simulink model "chip_route_circuit"  (R2025b)
settings: Solver=VariableStepAuto  StartTime=0.0  StopTime=10.0  RelTol=1e-3
libraries: fl_lib x44, nesl_utility x1
settings Model: Creator=97638  LastModifiedBy=97638

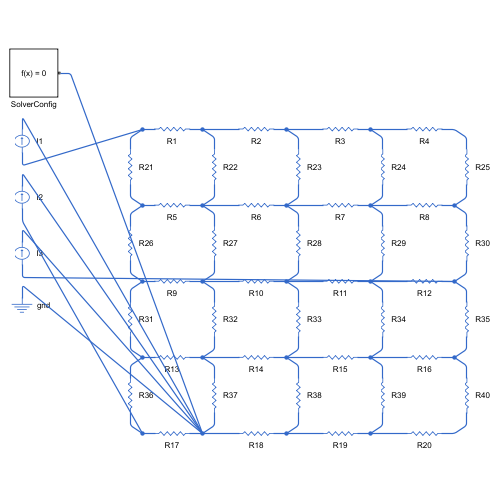
[thumbnail: Simulink's stored preview of the top-level diagram]
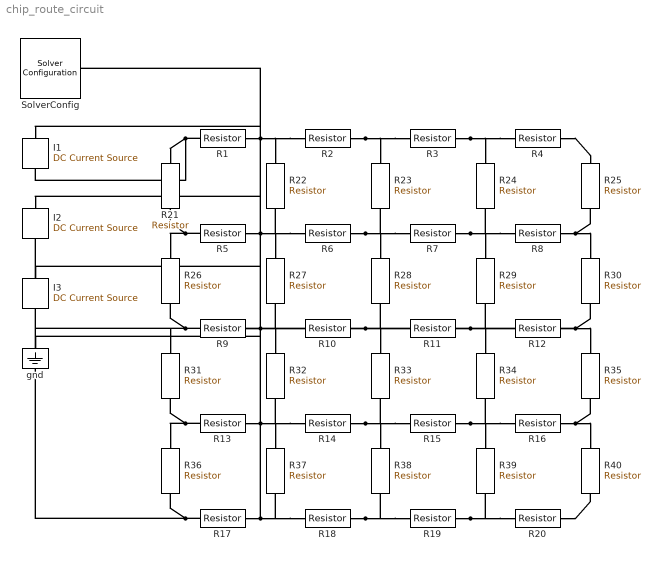
== system chip_route_circuit ==
  I1 : fl_lib/Electrical/Electrical Sources/DC Current Source  i0=1.0000 A
      settings: InternalSimscapePortConfiguration="{\"Bottom\":[],\"Left\":[{\"id\":\"p\",\"label\":\"\",\"type\":\"foundation.electrical.electrical\"}],\"Right\":[{\"id\":\"n\",\"label\":\"\",\"type\":\"foundation.electrical.electrical\"}],\"Top\":[]}"
  I2 : fl_lib/Electrical/Electrical Sources/DC Current Source  i0=1.0000 A
      settings: InternalSimscapePortConfiguration="{\"Bottom\":[],\"Left\":[{\"id\":\"p\",\"label\":\"\",\"type\":\"foundation.electrical.electrical\"}],\"Right\":[{\"id\":\"n\",\"label\":\"\",\"type\":\"foundation.electrical.electrical\"}],\"Top\":[]}"
  I3 : fl_lib/Electrical/Electrical Sources/DC Current Source  i0=-2.0000 A
      settings: InternalSimscapePortConfiguration="{\"Bottom\":[],\"Left\":[{\"id\":\"p\",\"label\":\"\",\"type\":\"foundation.electrical.electrical\"}],\"Right\":[{\"id\":\"n\",\"label\":\"\",\"type\":\"foundation.electrical.electrical\"}],\"Top\":[]}"
  R{1..40} (40 alike) : fl_lib/Electrical/Electrical Elements/Resistor  R=1.000000 Ohm  i_specify=off  i_priority=None  i=0 A  i_nominal_specify=off  i_nominal_value=1  i_nominal_unit=A  v_specify=off  v_priority=None  v=0 V  v_nominal_specify=off  v_nominal_value=1  v_nominal_unit=V
  SolverConfig : nesl_utility/Solver Configuration  PhysicalDomain=network_engine_domain  SubClassName=solver  LeftPortType=input  RightPortType=generic  Tones=[]  Harmonics=[]  SimulateNoise=off  Profile=off  UseLocalSampling=off  EnableSwitchedLinearOptims=on  FrequencyDomain=off  UseCCode=off  RelTol=0.001  AbsTol=0.001  MinStep=1e-09  ToWorkspace=off  RevertToSquareIcSolve=off  NumHomotopyIterations=100  PhasorMode=off  PhasorModeNumHarmonics=1  ConsistencySolver=NEWTON_XTOL_AFTER_FTOL  IndexReductionMethod=DerivativeReplacement  DoDC=off  ResidualTolerance=1e-09  ConsistencyTolSource=GLOBAL  ConsistencyAbsTol=0.001  ConsistencyRelTol=0.001  ConsistencyTolFactor=0.001  UseLocalSolver=off  LocalSolverChoice=NE_BACKWARD_EULER_ADVANCER  ResolveIndetEquations=on  FunctionEvalNumThread=1  LocalSolverSampleTime=0.001  DoFixedCost=off  MaxNonlinIter=3  MaxModeIter=2  ComputeImpulses=off  ImpulseIterations=2  LinearAlgebra=auto  LinearAlgebraNumThread=0  EquationFormulation=NE_TIME_EF  DelaysMemoryBudget=1024  AutomaticFiltering=on  FilteringTimeConstant=0.001  PartitionStorageMethod=AS_NEEDED  PartitionMemoryBudget=1024  PartitionMethod=ROBUST  MultibodyUseLocalSolver=off  MultibodyLocalSolverChoice=ODE1  MultibodyLocalSolverSampleTime=0.001
  gnd : fl_lib/Electrical/Electrical Elements/Electrical Reference
  connections:
  R21/LConn1 -- R1/LConn1 -- I1/RConn1
  R2/LConn1 -- R1/RConn1 -- R22/LConn1
  R3/LConn1 -- R2/RConn1 -- R23/LConn1
  R4/LConn1 -- R3/RConn1 -- R24/LConn1
  R4/RConn1 -- R25/LConn1
  R21/RConn1 -- R5/LConn1 -- R26/LConn1
  R6/LConn1 -- R5/RConn1 -- R22/RConn1 -- R27/LConn1
  R7/LConn1 -- R6/RConn1 -- R23/RConn1 -- R28/LConn1
  R8/LConn1 -- R7/RConn1 -- R24/RConn1 -- R29/LConn1
  R25/RConn1 -- R8/RConn1 -- R30/LConn1
  R26/RConn1 -- R9/LConn1 -- R31/LConn1
  R10/LConn1 -- R9/RConn1 -- R27/RConn1 -- R32/LConn1
  R11/LConn1 -- R10/RConn1 -- R28/RConn1 -- R33/LConn1
  R12/LConn1 -- R11/RConn1 -- R29/RConn1 -- R34/LConn1
  R30/RConn1 -- R12/RConn1 -- R35/LConn1 -- I3/RConn1
  R31/RConn1 -- R13/LConn1 -- R36/LConn1
  R14/LConn1 -- R13/RConn1 -- R32/RConn1 -- R37/LConn1
  R15/LConn1 -- R14/RConn1 -- R33/RConn1 -- R38/LConn1
  R16/LConn1 -- R15/RConn1 -- R34/RConn1 -- R39/LConn1
  R35/RConn1 -- R16/RConn1 -- R40/LConn1
  R36/RConn1 -- R17/LConn1 -- I2/RConn1
  R18/LConn1 -- R17/RConn1 -- R37/RConn1 -- gnd/LConn1 -- I1/LConn1 -- I2/LConn1 -- I3/LConn1 -- SolverConfig/RConn1
  R19/LConn1 -- R18/RConn1 -- R38/RConn1
  R20/LConn1 -- R19/RConn1 -- R39/RConn1
  R20/RConn1 -- R40/RConn1
